simulink model "Thyristor_Rectifier"  (R2021a)
settings: Solver=VariableStepAuto  StartTime=0.0  StopTime=10.0  RelTol=1e-3
undefined symbols (not defined in the file): D1, lagging, pulse
libraries: spsThreePhaseSeriesRLCBranchLib x2, spsPLL3phLib x1, spsPulseGeneratorThyristor6PulseLib x1, spsSeriesRLCBranchLib x1, spsThreePhaseParallelRLCLoadLib x1, spsThreePhaseVIMeasurementLib x1, spsThreePhaseSourceLib x1, spsUniversalBridgeLib x1, spspowerguiLib x1
settings Model: Creator=45276  LastModifiedBy=45276

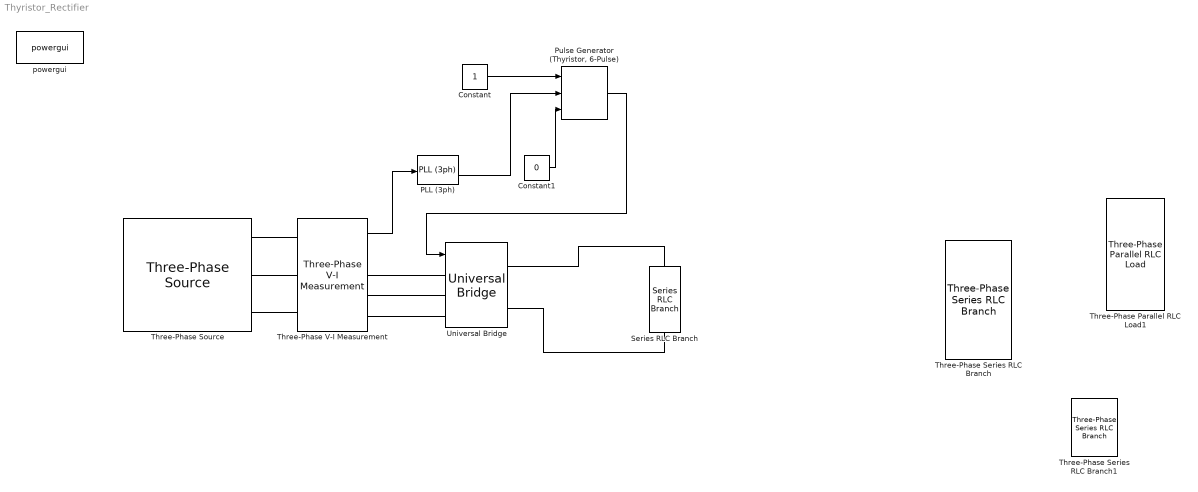
== system Thyristor_Rectifier ==
  Constant : Constant
  Constant1 : Constant  Value=0
  PLL (3ph) : spsPLL3phLib/PLL (3ph)  Fmin=45  Par_Init=[0, 60]  ParK=[180, 3200, 1]  TcD=1e-4  MaxRateChangeFreq=12  FilterCutOffFreq=25  Ts=0  AGC=on
  "Pulse Generator (Thyristor, 6-Pulse)" : spsPulseGeneratorThyristor6PulseLib/Pulse Generator (Thyristor, 6-Pulse)  GenType=6-pulse  Delta=D1 (lagging)  pwidth=60  Double_Pulse=off  Ts=0
      settings: SourceProductBaseCode=PS
  Series RLC Branch : spsSeriesRLCBranchLib/Series RLC Branch  LConnTagsString=__new0  RConnTagsString=__new0  BranchType=RLC  Resistance=1  Inductance=1e-3  SetiL0=off  InitialCurrent=0  Capacitance=1e-6  Setx0=off  InitialVoltage=0  Measurements=None
  Three-Phase Parallel RLC Load1 : spsThreePhaseParallelRLCLoadLib/Three-Phase Parallel RLC Load  LConnTagsString=A|B|C  Configuration=Y (grounded)  NominalVoltage=1000  Vabc=[1e3 1e3 1e3]  Vabcp=[1e3 1e3 1e3]  NominalFrequency=60  UnbalancedPower=off  ActivePower=10e3  InductivePower=100  CapacitivePower=100  Pabc=[10e3 9e3 11e3]  QLabc=[100 90 110]  QCabc=[100 90 110]  Pabcp=[10e3 9e3 11e3]  QLabcp=[100 90 110]  QCabcp=[100 90 110]  Measurements=None  LoadType=constant Z
  Three-Phase Series RLC Branch : spsThreePhaseSeriesRLCBranchLib/Three-Phase Series RLC Branch  LConnTagsString=A|B|C  RConnTagsString=A|B|C  BranchType=RLC  Resistance=1  Inductance=1e-3  Capacitance=1e-6  Measurements=None
  Three-Phase Series RLC Branch1 : spsThreePhaseSeriesRLCBranchLib/Three-Phase Series RLC Branch  LConnTagsString=A|B|C  RConnTagsString=A|B|C  BranchType=RLC  Resistance=1  Inductance=1e-3  Capacitance=1e-6  Measurements=None
  Three-Phase V-I Measurement : spsThreePhaseVIMeasurementLib/Three-Phase V-I Measurement  VoltageMeasurement=phase-to-ground  SetLabelV=off  LabelV=Vabc  Vpu=off  VpuLL=off  CurrentMeasurement=yes  SetLabelI=off  LabelI=Iabc  Ipu=off  Pbase=100e6  Vbase=500e3  OutputType=Complex  PhasorSimulation=off  PSBequivalent=0
  Three-Phase Source : spsThreePhaseSourceLib/Three-Phase Source  InternalConnection=Yg  VoltagePhases=off  Voltage=25e3  PhaseAngle=0  Voltage_phases=[25e3 25e3 25e3]/sqrt(3)  PhaseAngles_phases=[0 -120 +120]  Frequency=60  NonIdealSource=on  SpecifyImpedance=off  Resistance=0.8929  Inductance=16.58e-3  ShortCircuitLevel=100e6  BaseVoltage=25e3  XRratio=7  BusType=swing  Pref=10e3  Qref=0  Prefabc=[10e3, 10e3, 10e3]  Qrefabc=[0, 0, 0]  Qmin=-inf  Qmax=inf
  Universal Bridge : spsUniversalBridgeLib/Universal Bridge  Arms=3  SnubberResistance=1e5  SnubberCapacitance=inf  Device=Thyristors  Ron=1e-3  Lon=0  ForwardVoltages="[  0  0  ]"  ForwardVoltage=0  GTOparameters=[ 10e-6 , 20e-6 ]  IGBTparameters=[ 1e-6 , 2e-6 ]  Measurements=None  Measurements_2=None  converterType=Rectifier
  powergui : spspowerguiLib/powergui  Priority=1  SimulationMode=Continuous  SampleTime=50e-6  frequency=60  Iterations=50  frequencyindice=60  Pbase=100e6  ErrMax=1e-4  UnitsV=kV  UnitsW=MW  buscounter=0  FunctionMessages=off  echomessages=off  EnableUseOfTLC=off  CurrentSourceSwitches=off  DisableSnubberDevices=off  DisableRonSwitches=off  DisableVfSwitches=off  DisplayEquations=off  AutomaticDiscreteSolvers=off  SolverType=Tustin/Backward Euler (TBE)  Interpol=off  ExternalGateDelay=off  methode=off  Ts=100  x0status=blocks  SPID=on  SwTol=0  HookPort=off  NonlinearTolerance=1e-4  nMaxIteration=100  ContinueOnMaxIteration=off  RestoreLinks=warning  ResistiveCurrentMeasurement=off  Frange=[0:2:500]  Ylog=off  Xlog=on  ShowGrid=off  save=off  variable=ZData  structure=0  ZoomFFT=off  StartTime=0.0  cycles=1  DisplayStyle=1  fundamental=60  FreqAxis=off  MaxFrequency=1000  frequencyindicesteady=1  RmsSteady=1  display=off
  wires:
  Three-Phase V-I Measurement/1 -> PLL (3ph)/1
  PLL (3ph)/2 -> "Pulse Generator (Thyristor, 6-Pulse)"/2
  Constant1/1 -> "Pulse Generator (Thyristor, 6-Pulse)"/3
  Constant/1 -> "Pulse Generator (Thyristor, 6-Pulse)"/1
  "Pulse Generator (Thyristor, 6-Pulse)"/1 -> Universal Bridge/1
  connections:
  Three-Phase Source/RConn1 -- Three-Phase V-I Measurement/LConn1
  Three-Phase Source/RConn2 -- Three-Phase V-I Measurement/LConn2
  Three-Phase Source/RConn3 -- Three-Phase V-I Measurement/LConn3
  Universal Bridge/LConn1 -- Three-Phase V-I Measurement/RConn1
  Universal Bridge/LConn2 -- Three-Phase V-I Measurement/RConn2
  Universal Bridge/LConn3 -- Three-Phase V-I Measurement/RConn3
  Universal Bridge/RConn1 -- Series RLC Branch/LConn1
  Series RLC Branch/RConn1 -- Universal Bridge/RConn2
